simulink subsystem "attitude_plant"  (R2025a)
settings: Solver=VariableStepAuto  StartTime=0.0  StopTime=10.0  RelTol=1e-3
values from neighbouring files (symbols this model uses):
  b_pitch = 0    [drone_plant.m]    (also in plan_equations.m)
  b_roll = 0    [drone_plant.m]    (also in plan_equations.m)
  b_yaw = 0    [drone_plant.m]    (also in plan_equations.m)
  I_xx = 0.02    [drone_plant.m]    (also in plan_equations.m)
  I_yy = 0.02    [drone_plant.m]    (also in plan_equations.m)
  I_zz = 0.02    [drone_plant.m]    (also in plan_equations.m)
settings Model: Creator=flore  LastModifiedBy=flore

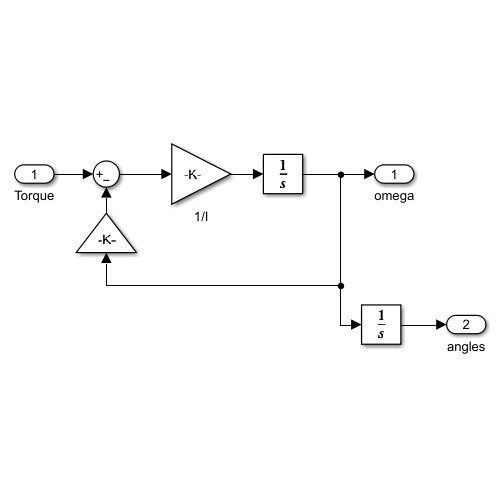
[thumbnail: Simulink's stored preview of the top-level diagram]
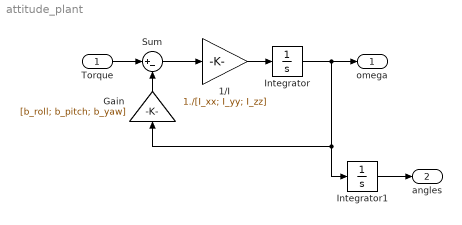
== system attitude_plant ==
  Torque : Inport
  1/I : Gain  Gain=1./[I_xx; I_yy; I_zz]
  Gain : Gain  Gain=[b_roll; b_pitch; b_yaw]
  Integrator : Integrator  InitialCondition=[0;0;0]
  Integrator1 : Integrator  InitialCondition=[0;0;0]
  Sum : Sum  Inputs=|+-
  omega : Outport
  angles : Outport  Port=2
  wires:
  Torque/1 -> Sum/1
  Gain/1 -> Sum/2
  Sum/1 -> 1/I/1
  1/I/1 -> Integrator/1
  Integrator/1 -> omega/1, Integrator1/1, Gain/1
  Integrator1/1 -> angles/1
